simulink model "Exp6"  (R2025b)
settings: Solver=VariableStepAuto  StartTime=0.0  StopTime=10.0  RelTol=1e-3
settings Model: Creator=SUBHASH  LastModifiedBy=SUBHASH

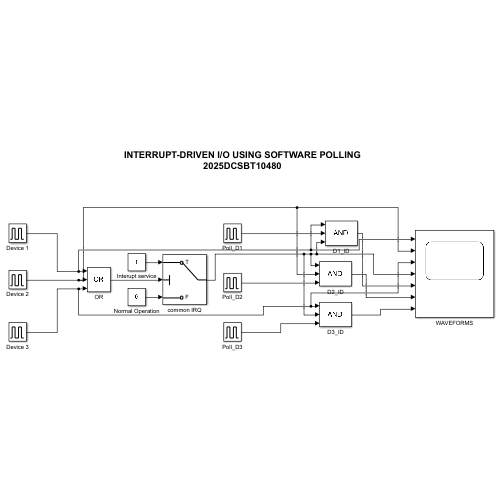
[thumbnail: Simulink's stored preview of the top-level diagram]
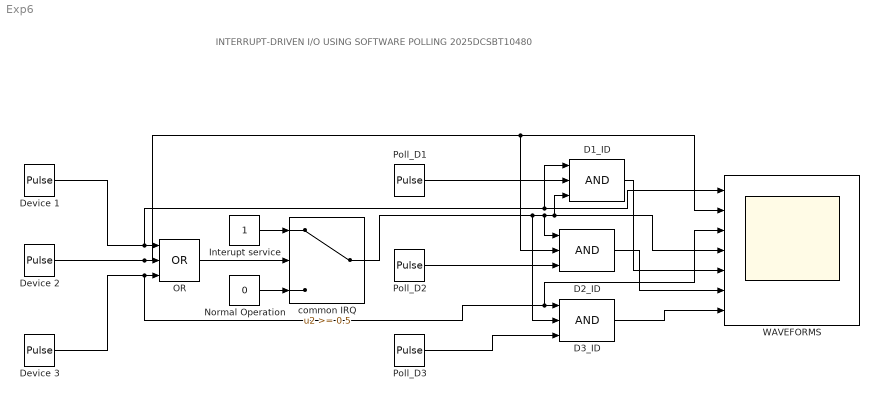
== system Exp6 ==
  note: INTERRUPT-DRIVEN I/O USING SOFTWARE POLLING
      | 2025DCSBT10480
  D1_ID : Logic  Inputs=3  AllPortsSameDT=off  OutDataTypeStr=boolean
  D2_ID : Logic  Inputs=3  AllPortsSameDT=off  OutDataTypeStr=boolean
  D3_ID : Logic  Inputs=3  AllPortsSameDT=off  OutDataTypeStr=boolean
  Device 1 : DiscretePulseGenerator  PulseType=Time based  Period=12  PulseWidth=10  PhaseDelay=2
  Device 2 : DiscretePulseGenerator  PulseType=Time based  Period=12  PulseWidth=10  PhaseDelay=4
  Device 3 : DiscretePulseGenerator  PulseType=Time based  Period=12  PulseWidth=10  PhaseDelay=6
  Interupt service : Constant
  Normal Operation : Constant  Value=0
  OR : Logic  Operator=OR  Inputs=3  AllPortsSameDT=off  OutDataTypeStr=boolean
  Poll_D1 : DiscretePulseGenerator  PulseType=Time based  Period=12  PulseWidth=5  PhaseDelay=2
  Poll_D2 : DiscretePulseGenerator  PulseType=Time based  Period=12  PulseWidth=5  PhaseDelay=4
  Poll_D3 : DiscretePulseGenerator  PulseType=Time based  Period=12  PulseWidth=5  PhaseDelay=6
  WAVEFORMS : Scope  NumInputPorts=7
      settings: TimeSpan=10  ActiveDisplayYMinimum=-0.12499999999999997  ActiveDisplayYMaximum=1.125
  common IRQ : Switch  Threshold=0.5  SaturateOnIntegerOverflow=off  InputSameDT=off
  wires:
  Device 1/1 -> D1_ID/1, WAVEFORMS/1, OR/1
  Device 2/1 -> D2_ID/2, WAVEFORMS/2, OR/2
  Device 3/1 -> WAVEFORMS/3, D3_ID/1, OR/3
  OR/1 -> common IRQ/2
  Normal Operation/1 -> common IRQ/3
  Interupt service/1 -> common IRQ/1
  D1_ID/1 -> WAVEFORMS/5
  D2_ID/1 -> WAVEFORMS/6
  D3_ID/1 -> WAVEFORMS/7
  Poll_D1/1 -> D1_ID/2
  Poll_D2/1 -> D2_ID/3
  Poll_D3/1 -> D3_ID/3
  common IRQ/1 -> D2_ID/1, D1_ID/3, WAVEFORMS/4, D3_ID/2
